simulink model "Lab8"  (R2023b)
settings: Solver=VariableStepAuto  StartTime=0.0  StopTime=100  RelTol=1e-3
settings Model: Creator=user  LastModifiedBy=user

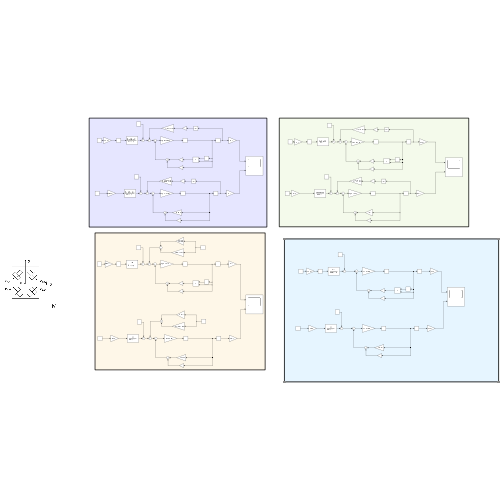
[thumbnail: Simulink's stored preview of the top-level diagram]
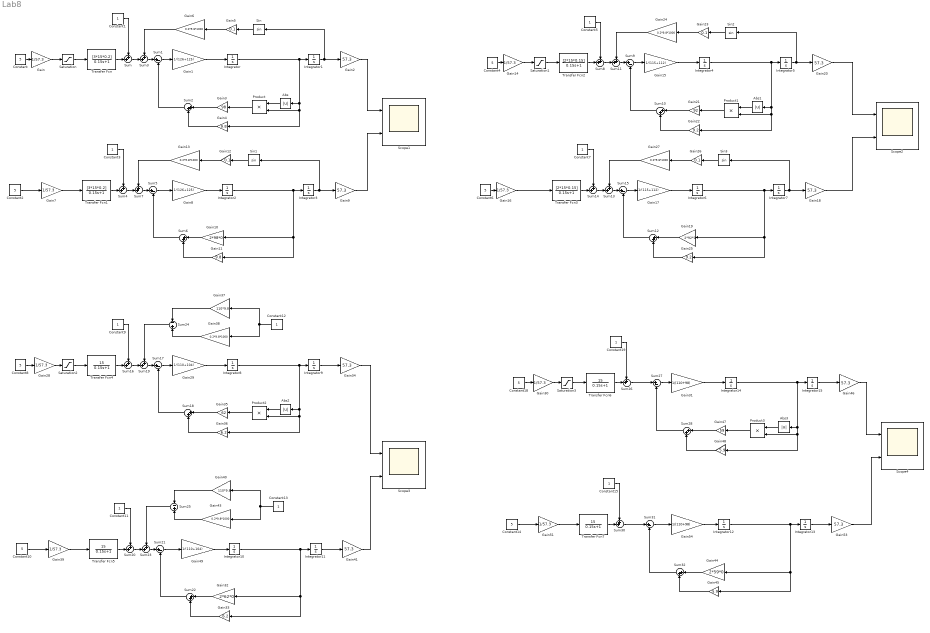
== system Lab8 ==
  Abs{,1..3} (4 alike) : Abs  SaturateOnIntegerOverflow=off
  Constant{,2,4,6,8,10,14,18} (8 alike) : Constant  Value=5
  Constant{1,3,5,7,9,11..13,15,19} (10 alike) : Constant
  Gain{,7,14,16,28,30,39,51} (8 alike) : Gain  Gain=1/57.3
  Gain1 : Gain  Gain=1/(126+125)
  Gain10 : Gain  Gain=2*98*0
  Gain11 : Gain  Gain=9.8
  Gain{5,12,23,26} (4 alike) : Gain  Gain=0.1
  Gain{6,13,24,27,38,43} (6 alike) : Gain  Gain=0.2*9.8*1000
  Gain15 : Gain  Gain=1/(115+112)
  Gain17 : Gain  Gain=1/(115+112)
  Gain{2,9,18,20,34,41,46,53} (8 alike) : Gain  Gain=57.3
  Gain19 : Gain  Gain=2*92*0
  Gain21 : Gain  Gain=92
  Gain22 : Gain  Gain=9.2
  Gain25 : Gain  Gain=9.2
  Gain29 : Gain  Gain=1/(110+104)
  Gain3 : Gain  Gain=98
  Gain31 : Gain  Gain=1/(110+98)
  Gain32 : Gain  Gain=2*62*0
  Gain33 : Gain  Gain=6.2
  Gain35 : Gain  Gain=62
  Gain36 : Gain  Gain=6.2
  Gain37 : Gain  Gain=110*9.8
  Gain4 : Gain  Gain=9.8
  Gain40 : Gain  Gain=110*9.8
  Gain44 : Gain  Gain=2*59*0
  Gain45 : Gain  Gain=5.9
  Gain47 : Gain  Gain=59
  Gain48 : Gain  Gain=5.9
  Gain49 : Gain  Gain=1/(110+104)
  Gain54 : Gain  Gain=1/(110+98)
  Gain8 : Gain  Gain=1/(126+125)
  Integrator{,1..15} (16 alike) : Integrator
  Product{,1..3} (4 alike) : Product
  Saturation{,1..3} (4 alike) : Saturate  UpperLimit=10  LowerLimit=-10
  Scope{1..4} (4 alike) : Scope  NumInputPorts=2
  Sin{,1..3} (4 alike) : Trigonometry
  Sum{,3..4,7..8,11,13..14,16,19..20,23,26,30} (14 alike) : Sum  Inputs=++|
  Sum{1,5,9,15,17,21,27,31} (8 alike) : Sum  Inputs=|+-
  Sum{2,6,10,12,18,22,28,32} (8 alike) : Sum  Inputs=|++
  Sum24 : Sum  Inputs=-|+
  Sum25 : Sum  Inputs=-|+
  Transfer Fcn : TransferFcn  Numerator=[3*15*0.2]  Denominator=[0.15 1]
  Transfer Fcn1 : TransferFcn  Numerator=[3*15*0.2]  Denominator=[0.15 1]
  Transfer Fcn2 : TransferFcn  Numerator=[2*15*0.15]  Denominator=[0.15 1]
  Transfer Fcn3 : TransferFcn  Numerator=[2*15*0.15]  Denominator=[0.15 1]
  Transfer Fcn{4..7} (4 alike) : TransferFcn  Numerator=[15]  Denominator=[0.15 1]
  wires:
  Constant/1 -> Gain/1
  Gain/1 -> Saturation/1
  Saturation/1 -> Transfer Fcn/1
  Transfer Fcn/1 -> Sum/2
  Constant1/1 -> Sum/1
  Sum1/1 -> Gain1/1
  Gain1/1 -> Integrator/1
  Integrator/1 -> Gain4/1, Product/2, Abs/1, Integrator1/1
  Integrator1/1 -> Sin/1, Gain2/1
  Abs/1 -> Product/1
  Product/1 -> Gain3/1
  Gain3/1 -> Sum2/1
  Sum2/1 -> Sum1/2
  Gain4/1 -> Sum2/2
  Sin/1 -> Gain5/1
  Gain5/1 -> Gain6/1
  Sum/1 -> Sum3/2
  Sum3/1 -> Sum1/1
  Gain6/1 -> Sum3/1
  Gain2/1 -> Scope1/1
  Gain9/1 -> Scope1/2
  Gain13/1 -> Sum7/1
  Sum7/1 -> Sum5/1
  Sum4/1 -> Sum7/2
  Gain12/1 -> Gain13/1
  Sin1/1 -> Gain12/1
  Gain11/1 -> Sum6/2
  Sum6/1 -> Sum5/2
  Gain10/1 -> Sum6/1
  Integrator2/1 -> Integrator3/1, Gain11/1, Gain10/1
  Integrator3/1 -> Sin1/1, Gain9/1
  Gain8/1 -> Integrator2/1
  Sum5/1 -> Gain8/1
  Constant3/1 -> Sum4/1
  Transfer Fcn1/1 -> Sum4/2
  Gain7/1 -> Transfer Fcn1/1
  Constant2/1 -> Gain7/1
  Gain23/1 -> Gain24/1
  Sum11/1 -> Sum9/1
  Gain20/1 -> Scope2/1
  Sin2/1 -> Gain23/1
  Gain24/1 -> Sum11/1
  Product1/1 -> Gain21/1
  Sum8/1 -> Sum11/2
  Integrator5/1 -> Sin2/1, Gain20/1
  Abs1/1 -> Product1/1
  Sum10/1 -> Sum9/2
  Transfer Fcn2/1 -> Sum8/2
  Sum9/1 -> Gain15/1
  Saturation1/1 -> Transfer Fcn2/1
  Constant5/1 -> Sum8/1
  Integrator4/1 -> Gain22/1, Product1/2, Abs1/1, Integrator5/1
  Gain21/1 -> Sum10/1
  Gain15/1 -> Integrator4/1
  Gain22/1 -> Sum10/2
  Gain14/1 -> Saturation1/1
  Constant4/1 -> Gain14/1
  Constant6/1 -> Gain16/1
  Gain25/1 -> Sum12/2
  Gain19/1 -> Sum12/1
  Gain17/1 -> Integrator6/1
  Constant7/1 -> Sum14/1
  Transfer Fcn3/1 -> Sum14/2
  Sum12/1 -> Sum15/2
  Gain16/1 -> Transfer Fcn3/1
  Sum15/1 -> Gain17/1
  Integrator7/1 -> Sin3/1, Gain18/1
  Sin3/1 -> Gain26/1
  Gain18/1 -> Scope2/2
  Integrator6/1 -> Gain25/1, Gain19/1, Integrator7/1
  Sum13/1 -> Sum15/1
  Gain27/1 -> Sum13/1
  Gain26/1 -> Gain27/1
  Sum14/1 -> Sum13/2
  Gain34/1 -> Scope3/1
  Gain39/1 -> Transfer Fcn5/1
  Integrator9/1 -> Gain34/1
  Sum19/1 -> Sum17/1
  Constant10/1 -> Gain39/1
  Integrator10/1 -> Integrator11/1, Gain33/1, Gain32/1
  Constant11/1 -> Sum20/1
  Integrator11/1 -> Gain41/1
  Sum20/1 -> Sum23/2
  Gain32/1 -> Sum22/1
  Sum22/1 -> Sum21/2
  Sum23/1 -> Sum21/1
  Product2/1 -> Gain35/1
  Transfer Fcn5/1 -> Sum20/2
  Sum16/1 -> Sum19/2
  Abs2/1 -> Product2/1
  Sum18/1 -> Sum17/2
  Transfer Fcn4/1 -> Sum16/2
  Sum17/1 -> Gain29/1
  Saturation2/1 -> Transfer Fcn4/1
  Constant9/1 -> Sum16/1
  Integrator8/1 -> Gain36/1, Product2/2, Abs2/1, Integrator9/1
  Gain33/1 -> Sum22/2
  Gain35/1 -> Sum18/1
  Gain29/1 -> Integrator8/1
  Gain36/1 -> Sum18/2
  Gain28/1 -> Saturation2/1
  Constant8/1 -> Gain28/1
  Gain41/1 -> Scope3/2
  Sum21/1 -> Gain49/1
  Constant12/1 -> Gain38/1, Gain37/1
  Gain37/1 -> Sum24/1
  Gain38/1 -> Sum24/2
  Sum24/1 -> Sum19/1
  Gain49/1 -> Integrator10/1
  Gain43/1 -> Sum25/2
  Gain40/1 -> Sum25/1
  Constant13/1 -> Gain40/1, Gain43/1
  Sum25/1 -> Sum23/1
  Gain54/1 -> Integrator12/1
  Sum31/1 -> Gain54/1
  Gain53/1 -> Scope4/2
  Constant18/1 -> Gain30/1
  Gain30/1 -> Saturation3/1
  Gain48/1 -> Sum28/2
  Gain31/1 -> Integrator14/1
  Gain47/1 -> Sum28/1
  Gain45/1 -> Sum32/2
  Integrator14/1 -> Integrator15/1, Abs3/1, Product3/2, Gain48/1
  Constant19/1 -> Sum26/1
  Saturation3/1 -> Transfer Fcn6/1
  Sum27/1 -> Gain31/1
  Transfer Fcn6/1 -> Sum26/2
  Sum28/1 -> Sum27/2
  Abs3/1 -> Product3/1
  Transfer Fcn7/1 -> Sum30/2
  Product3/1 -> Gain47/1
  Sum30/1 -> Sum31/1
  Sum32/1 -> Sum31/2
  Gain44/1 -> Sum32/1
  Integrator13/1 -> Gain53/1
  Constant15/1 -> Sum30/1
  Integrator12/1 -> Gain44/1, Gain45/1, Integrator13/1
  Constant14/1 -> Gain51/1
  Integrator15/1 -> Gain46/1
  Gain51/1 -> Transfer Fcn7/1
  Gain46/1 -> Scope4/1
  Sum26/1 -> Sum27/1
